simulink model "gyroerr_test_drvr"  (Simulink 4.00)
settings: Solver=ode45  StartTime=0.0  StopTime=1  RelTol=1e-3
undefined symbols (not defined in the file or in its folder): CBL, dcm2pitch, dcm2roll, dcm2yaw, skew
settings Model: Creator=mcar  LastModifiedBy=mcar  BlockReductionOpt=off

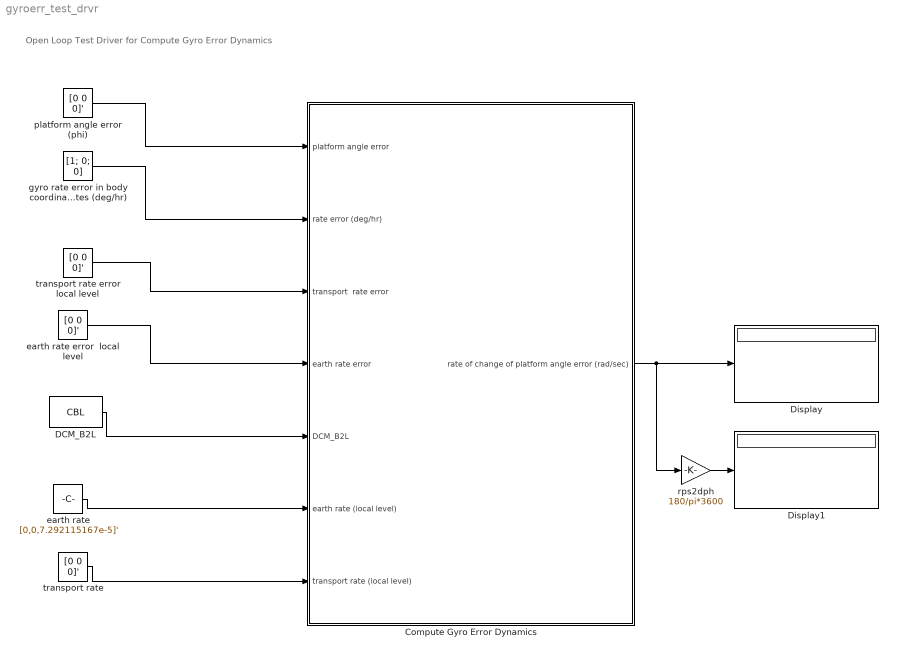
== system gyroerr_test_drvr ==
  note: Open Loop Test Driver
      | for
      | Compute Gyro Error Dynamics
  Compute Gyro Error Dynamics : Subsystem
      settings: RTWFcnNameOpts=Auto  RTWFileNameOpts=Auto
  DCM_B2L : Constant  Value=CBL  VectorParams1D=off
  Display : Display
  Display1 : Display
  earth rate : Constant  Value=[0,0,7.292115167e-5]'  VectorParams1D=off
  earth rate error  local level : Constant  Value=[0 0 0]'  VectorParams1D=off
  gyro rate error in body coordinates (deg/hr) : Constant  Value=[1; 0; 0]  VectorParams1D=off
  platform angle error (phi) : Constant  Value=[0 0 0]'  VectorParams1D=off
  rps2dph : Gain  Gain=180/pi*3600  Multiplication=Element-wise(K.*u)  SaturateOnIntegerOverflow=on
  transport rate : Constant  Value=[0 0 0]'  VectorParams1D=off
  transport rate error local level : Constant  Value=[0 0 0]'  VectorParams1D=off
  wires:
  platform angle error (phi)/1 -> Compute Gyro Error Dynamics/1(platform angle error)
  transport rate error local level/1 -> Compute Gyro Error Dynamics/3(transport  rate error)
  earth rate error  local level/1 -> Compute Gyro Error Dynamics/4(earth rate error)
  DCM_B2L/1 -> Compute Gyro Error Dynamics/5(DCM_B2L)
  transport rate/1 -> Compute Gyro Error Dynamics/7(transport rate (local level))
  earth rate/1 -> Compute Gyro Error Dynamics/6(earth rate (local level))
  gyro rate error in body coordinates (deg/hr)/1 -> Compute Gyro Error Dynamics/2(rate error (deg/hr))
  Compute Gyro Error Dynamics/1(rate of change of platform angle error (rad/sec)) -> Display/1, rps2dph/1
  rps2dph/1 -> Display1/1

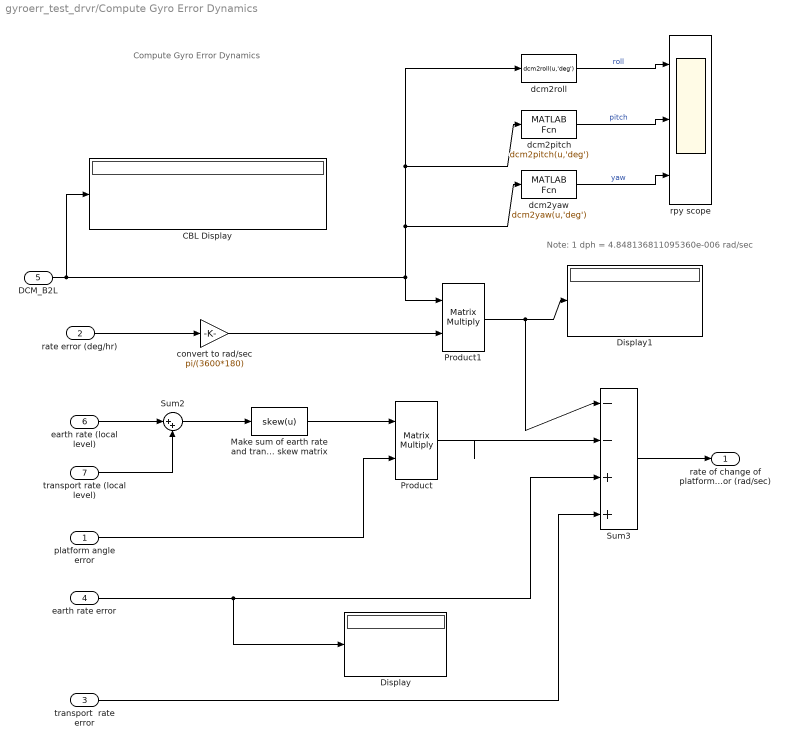
== system gyroerr_test_drvr/Compute Gyro Error Dynamics ==
  note: Compute Gyro Error Dynamics
  note: Note: 1 dph = 4.848136811095360e-006 rad/sec
  platform angle error : Inport  Port=1
  rate error (deg/hr) : Inport  Port=2
  transport  rate error : Inport  Port=3
  earth rate error : Inport  Port=4
  DCM_B2L : Inport  Port=5
  earth rate (local level) : Inport  Port=6
  transport rate (local level) : Inport  Port=7
  CBL Display : Display
      settings: Format=short_e
  Display : Display
      settings: Format=short
  Display1 : Display
  Make sum of earth rate and transport rates  a skew matrix : MATLABFcn  MATLABFcn=skew(u)  OutputDimensions=-1  OutputSignalType=auto  Output1D=off
  Product : Product  Inputs=2  Multiplication=Matrix(*)  SaturateOnIntegerOverflow=on
  Product1 : Product  Inputs=2  Multiplication=Matrix(*)  SaturateOnIntegerOverflow=on
  Sum2 : Sum  Inputs=|++  SaturateOnIntegerOverflow=on
  Sum3 : Sum  Inputs=|--++  SaturateOnIntegerOverflow=on
  convert to rad/sec : Gain  Gain=pi/(3600*180)  Multiplication=Element-wise(K.*u)  SaturateOnIntegerOverflow=on
  dcm2pitch : MATLABFcn  MATLABFcn=dcm2pitch(u,'deg')  OutputDimensions=-1  OutputSignalType=auto  Output1D=off
  dcm2roll : MATLABFcn  MATLABFcn=dcm2roll(u,'deg')  OutputDimensions=-1  OutputSignalType=auto  Output1D=off
  dcm2yaw : MATLABFcn  MATLABFcn=dcm2yaw(u,'deg')  OutputDimensions=-1  OutputSignalType=auto  Output1D=off
  rpy scope : Scope  NumInputPorts=3
      settings: TimeRange=10  YMin=-1~-1~-1  YMax=1~1~1  SaveToWorkspace=off  SaveName=ScopeData2  LimitDataPoints=on  MaxDataPoints=10000
  rate of change of platform angle error (rad/sec) : Outport  Port=1
  wires:
  platform angle error/1 -> Product/2
  Sum2/1 -> Make sum of earth rate and transport rates  a skew matrix/1
  rate error (deg/hr)/1 -> convert to rad/sec/1
  Product1/1 -> Sum3/1, Display1/1
  Sum3/1 -> rate of change of platform angle error (rad/sec)/1
  transport  rate error/1 -> Sum3/4
  earth rate error/1 -> Sum3/3, Display/1
  DCM_B2L/1 -> Product1/1, dcm2yaw/1, dcm2pitch/1, dcm2roll/1, CBL Display/1
  earth rate (local level)/1 -> Sum2/1
  transport rate (local level)/1 -> Sum2/2
  Product/1 -> Sum3/2
  convert to rad/sec/1 -> Product1/2
  Make sum of earth rate and transport rates  a skew matrix/1 -> Product/1
  dcm2roll/1 -> rpy scope/1  "roll"
  dcm2pitch/1 -> rpy scope/2  "pitch"
  dcm2yaw/1 -> rpy scope/3  "yaw"
